simulink model "rand_walk"  (Simulink 4.00)
settings: Solver=ode45  StartTime=0.0  StopTime=100.0  RelTol=1e-3
libraries: simulink_extras x2, simulink3 x1
settings Model: Creator=mcar  LastModifiedBy=mcar  BlockReductionOpt=off

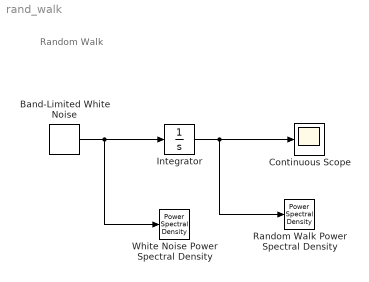
== system rand_walk ==
  note: Random Walk
  Band-Limited White Noise : simulink3/Sources/Band-Limited White Noise  Cov=[1]  Ts=0.01  seed=[23341]
  Continuous Scope : Scope
      settings: TimeRange=100  YMin=-3  YMax=4  SaveToWorkspace=off  SaveName=ScopeData  LimitDataPoints=on  MaxDataPoints=5000
  Integrator : Integrator  ExternalReset=none  InitialConditionSource=internal  InitialCondition=0  LimitOutput=off  UpperSaturationLimit=inf  LowerSaturationLimit=-inf  ShowSaturationPort=off  ShowStatePort=off  AbsoluteTolerance=auto
  Random Walk Power Spectral Density : simulink_extras/Additional Sinks/Power Spectral Density  npts=128  fftpts=512  HowOften=64  sampleT=0.1
  White Noise Power Spectral Density : simulink_extras/Additional Sinks/Power Spectral Density  npts=256  fftpts=512  HowOften=128  sampleT=0.01
  wires:
  Band-Limited White Noise/1 -> Integrator/1, White Noise Power Spectral Density/1
  Integrator/1 -> Continuous Scope/1, Random Walk Power Spectral Density/1
